simulink model "SYSTEM_MODEL_param_RAMP_SOC"  (R2024a)
settings: Solver=ode45  StartTime=0.0  StopTime=0.5  RelTol=1e-3
undefined symbols (not defined in the file): Cdc, Cf, Co, Dlim, Fsw, Io_max, Ion, kib, kii, kiv, Kmod, kpb, kpi, kpv, L, Lch, Lf, Lithium, Lt, R, Rf, V_grid, Vcv, Vdc
libraries: spsIGBTDiodeLib x7, spsSeriesRLCBranchLib x5, slpidlib x5, spsThreePhaseSeriesRLCBranchLib x3, spsCurrentMeasurementLib x2, spsVoltageMeasurementLib x2, spsabctodq0Lib x2, simulink x1, spsIGBTLib x1, spsPWMGeneratorDCDCLib x1, spsBatteryLib x1, spsPLL3phLib x1
settings Model: Creator=devashishraj  LastModifiedBy=Monz
settings DebuggingCC: UnconnectedInputMsg=warning  UnconnectedOutputMsg=warning  UnconnectedLineMsg=warning
settings ModelReferenceCC: EnableRefExpFcnMdlSchedulingChecks=on
settings RTWCC: GPUComputeCapability=3.5  DLArmComputeVersion=19.05

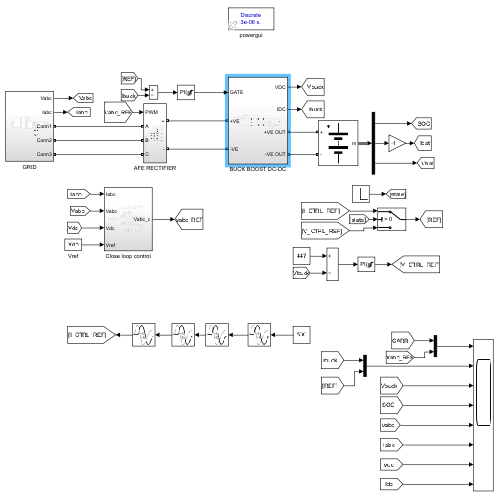
[thumbnail: Simulink's stored preview of the top-level diagram]
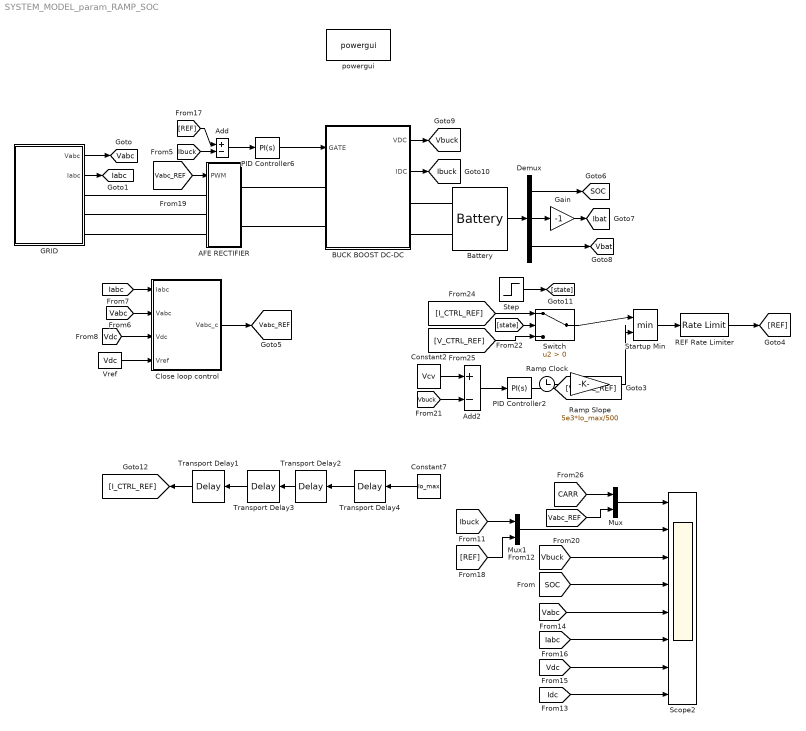
== system SYSTEM_MODEL_param_RAMP_SOC ==
  AFE RECTIFIER : Subsystem
  Add : Sum  Inputs=+-
  Add2 : Sum  Inputs=+-
  BUCK BOOST DC-DC : Subsystem
  Battery : spsBatteryLib/Battery  BatType=Lithium-Ion  ShowTempParam=off  ThermalPreset=no  ShowAgeParam=off  NomV=400  NomQ=250  SOC=SOC0  Batt_Tr=1  PresetModel=on  MaxQ=250  MinV=300  FullV=465.5949  Dis_rate=108.6957  R=0.016  Normal_OP=226.087  expZone="[432.1543      12.28261]"  current=[6.5 13 32.5]  Units=Time  Tci=20  NomT=20  T2=-30  MaxQ2=4.8  FullV2=7.1  Normal_OP2=5.655  expZone2="[6.58           1]"  Rca=0.6  ti=2000  Dp=0  Neq0=0  Tsim=1e6  Ta1=25  Qeol=5.4*0.9  Reol=0.013333*1.2  Char_age=[2.3478, 3]  Dis_age=[2.3478, 10]  N1=1500  N2=10500  N3=1000  N4=1400  Ta2=45  N5=950
  Close loop control : Subsystem
  Constant2 : Constant  Value=Vcv  SampleTime=2e-6
  Constant7 : Constant  Value=Io_max  SampleTime=2e-6
  Demux : Demux  Outputs=3
  GRID : Subsystem
  Gain : Gain  Gain=-1
  Mux : Mux  Inputs=2
  Mux1 : Mux  Inputs=2
  PID Controller2 : slpidlib/PID Controller  Controller=PI  Form=Parallel  TimeDomain=Continuous-time  UseExternalTs=off  SampleTime=-1  IntegratorMethod=Forward Euler  FilterMethod=Forward Euler  ControllerParametersSource=internal  P=0.75  I=50  UseKiTs=off  D=0  UseExternalDerivativeSource=off  N=100  UseFilter=on  TunerSelectOption=Transfer Function Based (PID Tuner App)  ZeroCross=off  InitialConditionSource=internal  InitialConditionForIntegrator=0  InitialConditionForFilter=0  DifferentiatorICPrevScaledInput=0  ExternalReset=none  TrackingMode=off  Kt=1  LimitOutput=on  SatLimitsSource=internal  UpperSaturationLimit=Io_max  LowerSaturationLimit=0  LinearizeAsGain=on  AntiWindupMode=clamping  Kb=1  LimitIntegrator=off  UpperIntegratorSaturationLimit=inf  LowerIntegratorSaturationLimit=-inf  POutMin=[]  POutMax=[]  IOutMin=[]  IOutMax=[]  DOutMin=[]  DOutMax=[]  NOutMin=[]  NOutMax=[]  SumOutMin=[]  SumOutMax=[]  SaturationOutMin=[]  SaturationOutMax=[]  PParamMin=[]  PParamMax=[]  IParamMin=[]  IParamMax=[]  DParamMin=[]  DParamMax=[]  NParamMin=[]  NParamMax=[]  KbParamMin=[]  KbParamMax=[]  KtParamMin=[]  KtParamMax=[]  KbOutMin=[]  KbOutMax=[]  KtOutMin=[]  KtOutMax=[]  IntegratorOutMin=[]  IntegratorOutMax=[]  FilterOutMin=[]  FilterOutMax=[]  SumI1OutMin=[]  SumI1OutMax=[]  SumI2OutMin=[]  SumI2OutMax=[]  SumI3OutMin=[]  SumI3OutMax=[]  SumI4OutMin=[]  SumI4OutMax=[]  SumDOutMin=[]  SumDOutMax=[]  DifferentiatorOutMin=[]  DifferentiatorOutMax=[]  FilterDiffOutCoefMin=[]  FilterDiffOutCoefMax=[]  ReciprocalOutMin=[]  ReciprocalOutMax=[]  SumDenOutMin=[]  SumDenOutMax=[]  SumNumOutMin=[]  SumNumOutMax=[]  DivideOutMin=[]  DivideOutMax=[]  UdiffTsProdOutMin=[]  UdiffTsProdOutMax=[]  NTsProdOutMin=[]  NTsProdOutMax=[]  UintegralTsProdOutMin=[]  UintegralTsProdOutMax=[]  UngainTsProdOutMin=[]  UngainTsProdOutMax=[]  ClampingZeroOutDataTypeStr=Inherit: Inherit via back propagation  ClampingZeroOutMin=[]  ClampingZeroOutMax=[]  FilterDenConstantOutDataTypeStr=Inherit: Inherit via back propagation  FilterDenConstantOutMin=[]  FilterDenConstantOutMax=[]  PCopyOutDataTypeStr=Inherit: Inherit via back propagation  PCopyOutMin=[]  PCopyOutMax=[]  NCopyOutDataTypeStr=Inherit: Inherit via back propagation  NCopyOutMin=[]  NCopyOutMax=[]  IntegratorContinuousStateAttributes=''  IntegratorStateMustResolveToSignalObject=off  IntegratorRTWStateStorageClass=Auto  FilterContinuousStateAttributes=''  FilterStateMustResolveToSignalObject=off  FilterRTWStateStorageClass=Auto  ParallelPVariant=InternalParameters  IdealPVariant=Disabled  IVariant=InternalParameters  DVariant=Disabled  IntegratorVariant=Continuous  SatVariant=Enabled  AWVariant=ContClampingParallel  PCopyVariant=Disabled  TRVariant=Disabled  FdbkBlocksVariant=Forward  IdealPFdbkVariant=Disabled  SatFdbkVariant=Disabled  DerivativeFilterVariant=Disabled  NVariant=Disabled  NCopyVariant=Disabled_SignalSpec  FilterICVariant=Disabled  IntegratorICVariant=InternalICs  ExternalResetVariant=Disabled  TRSumVariant=Passthrough  SumFdbkVariant=Disabled  SumVariant=Sum_PI  TsampFilterVariant=InternalTs  TsampNgainVariant=Passthrough  TsampIntegralVariant=Disabled_SignalSpec  ExternalSaturationOutDataTypeStr=Inherit: Same as second input  DerivativeSourceVariant=Disabled
  PID Controller6 : slpidlib/PID Controller  Controller=PI  Form=Parallel  TimeDomain=Continuous-time  UseExternalTs=off  SampleTime=-1  IntegratorMethod=Forward Euler  FilterMethod=Forward Euler  ControllerParametersSource=internal  P=kpb  I=kib  UseKiTs=off  D=0  UseExternalDerivativeSource=off  N=100  UseFilter=on  TunerSelectOption=Transfer Function Based (PID Tuner App)  ZeroCross=off  InitialConditionSource=internal  InitialConditionForIntegrator=0  InitialConditionForFilter=0  DifferentiatorICPrevScaledInput=0  ExternalReset=none  TrackingMode=off  Kt=1  LimitOutput=on  SatLimitsSource=internal  UpperSaturationLimit=Dlim  LowerSaturationLimit=0  LinearizeAsGain=on  AntiWindupMode=clamping  Kb=1  LimitIntegrator=off  UpperIntegratorSaturationLimit=inf  LowerIntegratorSaturationLimit=-inf  POutMin=[]  POutMax=[]  IOutMin=[]  IOutMax=[]  DOutMin=[]  DOutMax=[]  NOutMin=[]  NOutMax=[]  SumOutMin=[]  SumOutMax=[]  SaturationOutMin=[]  SaturationOutMax=[]  PParamMin=[]  PParamMax=[]  IParamMin=[]  IParamMax=[]  DParamMin=[]  DParamMax=[]  NParamMin=[]  NParamMax=[]  KbParamMin=[]  KbParamMax=[]  KtParamMin=[]  KtParamMax=[]  KbOutMin=[]  KbOutMax=[]  KtOutMin=[]  KtOutMax=[]  IntegratorOutMin=[]  IntegratorOutMax=[]  FilterOutMin=[]  FilterOutMax=[]  SumI1OutMin=[]  SumI1OutMax=[]  SumI2OutMin=[]  SumI2OutMax=[]  SumI3OutMin=[]  SumI3OutMax=[]  SumI4OutMin=[]  SumI4OutMax=[]  SumDOutMin=[]  SumDOutMax=[]  DifferentiatorOutMin=[]  DifferentiatorOutMax=[]  FilterDiffOutCoefMin=[]  FilterDiffOutCoefMax=[]  ReciprocalOutMin=[]  ReciprocalOutMax=[]  SumDenOutMin=[]  SumDenOutMax=[]  SumNumOutMin=[]  SumNumOutMax=[]  DivideOutMin=[]  DivideOutMax=[]  UdiffTsProdOutMin=[]  UdiffTsProdOutMax=[]  NTsProdOutMin=[]  NTsProdOutMax=[]  UintegralTsProdOutMin=[]  UintegralTsProdOutMax=[]  UngainTsProdOutMin=[]  UngainTsProdOutMax=[]  ClampingZeroOutDataTypeStr=Inherit: Inherit via back propagation  ClampingZeroOutMin=[]  ClampingZeroOutMax=[]  FilterDenConstantOutDataTypeStr=Inherit: Inherit via back propagation  FilterDenConstantOutMin=[]  FilterDenConstantOutMax=[]  PCopyOutDataTypeStr=Inherit: Inherit via back propagation  PCopyOutMin=[]  PCopyOutMax=[]  NCopyOutDataTypeStr=Inherit: Inherit via back propagation  NCopyOutMin=[]  NCopyOutMax=[]  IntegratorContinuousStateAttributes=''  IntegratorStateMustResolveToSignalObject=off  IntegratorRTWStateStorageClass=Auto  FilterContinuousStateAttributes=''  FilterStateMustResolveToSignalObject=off  FilterRTWStateStorageClass=Auto  ParallelPVariant=InternalParameters  IdealPVariant=Disabled  IVariant=InternalParameters  DVariant=Disabled  IntegratorVariant=Continuous  SatVariant=Enabled  AWVariant=ContClampingParallel  PCopyVariant=Disabled  TRVariant=Disabled  FdbkBlocksVariant=Forward  IdealPFdbkVariant=Disabled  SatFdbkVariant=Disabled  DerivativeFilterVariant=Disabled  NVariant=Disabled  NCopyVariant=Disabled_SignalSpec  FilterICVariant=Disabled  IntegratorICVariant=InternalICs  ExternalResetVariant=Disabled  TRSumVariant=Passthrough  SumFdbkVariant=Disabled  SumVariant=Sum_PI  TsampFilterVariant=InternalTs  TsampNgainVariant=Passthrough  TsampIntegralVariant=Disabled_SignalSpec  ExternalSaturationOutDataTypeStr=Inherit: Same as second input  DerivativeSourceVariant=Disabled
  Scope2 : Scope  NumInputPorts=8
  Step : Step  Time=0.4  Before=1  After=0  SampleTime=0
  Switch : Switch  Criteria=u2 > Threshold  SaturateOnIntegerOverflow=off  InputSameDT=off
  Transport Delay1 : TransportDelay  DelayTime=0.07  InitialOutput=0.4*Io_max
  Transport Delay2 : TransportDelay  DelayTime=0.07  InitialOutput=0.8*Io_max
  Transport Delay3 : TransportDelay  DelayTime=0.07  InitialOutput=0.6*Io_max
  Transport Delay4 : TransportDelay  DelayTime=0.07  InitialOutput=Io_max
  Vref : Constant  Value=Vdc
  powergui : spspowerguiLib/powergui  Priority=1  SimulationMode=Discrete  SampleTime=3e-6  frequency=60  Iterations=50  frequencyindice=0  Pbase=100e6  ErrMax=1e-4  UnitsV=kV  UnitsW=MW  buscounter=0  FunctionMessages=off  echomessages=off  EnableUseOfTLC=off  CurrentSourceSwitches=off  DisableSnubberDevices=off  DisableRonSwitches=off  DisableVfSwitches=off  DisplayEquations=off  AutomaticDiscreteSolvers=off  SolverType=Tustin/Backward Euler (TBE)  Interpol=off  ExternalGateDelay=off  methode=off  Ts=100  x0status=blocks  SPID=on  SwTol=0  HookPort=off  NonlinearTolerance=1e-4  nMaxIteration=100  ContinueOnMaxIteration=off  RestoreLinks=warning  ResistiveCurrentMeasurement=off  Frange=[0:2:500]  Ylog=off  Xlog=on  ShowGrid=off  save=off  variable=ZData  structure=0  ZoomFFT=off  StartTime=0.0  cycles=1  DisplayStyle=1  fundamental=60  FreqAxis=off  MaxFrequency=1000  frequencyindicesteady=1  RmsSteady=1  display=off
  Ramp Clock : Clock
  Ramp Slope : Gain  Gain=5e3*Io_max/500
  Startup Min : MinMax  Inputs=2
  REF Rate Limiter : RateLimiter  RisingSlewLimit=5e3*Io_max/500  FallingSlewLimit=-(5e3*Io_max/500)
  tag scope: Iabc=global, Ibat=global, Ibuck=global, SOC=global, Vabc=global, Vabc_REF=global, Vbat=global, Vbuck=global
  wires:
  GRID/1(Vabc) -> [Vabc]
  GRID/2(Iabc) -> [Iabc]
  [Iabc] -> Close loop control/1(Iabc)
  [Vabc] -> Close loop control/2(Vabc)
  Battery/1 -> Demux/1
  Demux/2 -> Gain/1
  Demux/1 -> [SOC]
  Gain/1 -> [Ibat]
  Demux/3 -> [Vbat]
  [CARR] -> Mux/1
  Mux/1 -> Scope2/1
  Close loop control/1(Vabc_c) -> [Vabc_REF]
  [Ibuck] -> Add/2
  Add/1 -> PID Controller6/1
  [Ibuck] -> Mux1/1
  Mux1/1 -> Scope2/2
  [SOC] -> Scope2/4
  [Idc] -> Scope2/8
  [Vabc] -> Scope2/5
  [Iabc] -> Scope2/6
  [REF] -> Add/1
  [REF] -> Mux1/2
  [Vabc_REF] -> AFE RECTIFIER/1(PWM)
  [Vabc_REF] -> Mux/2
  PID Controller6/1 -> BUCK BOOST DC-DC/1(GATE)
  BUCK BOOST DC-DC/1(VDC) -> [Vbuck]
  BUCK BOOST DC-DC/2(IDC) -> [Ibuck]
  [state] -> Switch/2
  [V_CTRL_REF] -> Switch/3
  [I_CTRL_REF] -> Switch/1
  Switch/1 -> Startup Min/1
  [Vdc] -> Close loop control/3(Vdc)
  Vref/1 -> Close loop control/4(Vref)
  PID Controller2/1 -> [V_CTRL_REF]
  Add2/1 -> PID Controller2/1
  [Vbuck] -> Add2/2
  Constant2/1 -> Add2/1
  Step/1 -> [state]
  [Vdc] -> Scope2/7
  Constant7/1 -> Transport Delay4/1
  Transport Delay1/1 -> [I_CTRL_REF]
  Transport Delay2/1 -> Transport Delay3/1
  Transport Delay3/1 -> Transport Delay1/1
  Transport Delay4/1 -> Transport Delay2/1
  [Vbuck] -> Scope2/3
  Ramp Clock/1 -> Ramp Slope/1
  Ramp Slope/1 -> Startup Min/2
  Startup Min/1 -> REF Rate Limiter/1
  REF Rate Limiter/1 -> [REF]
  connections:
  GRID/RConn1 -- AFE RECTIFIER/LConn1
  GRID/RConn2 -- AFE RECTIFIER/LConn2
  GRID/RConn3 -- AFE RECTIFIER/LConn3
  BUCK BOOST DC-DC/LConn1 -- AFE RECTIFIER/RConn1
  AFE RECTIFIER/RConn2 -- BUCK BOOST DC-DC/LConn2
  Battery/LConn1 -- BUCK BOOST DC-DC/RConn1
  Battery/LConn2 -- BUCK BOOST DC-DC/RConn2

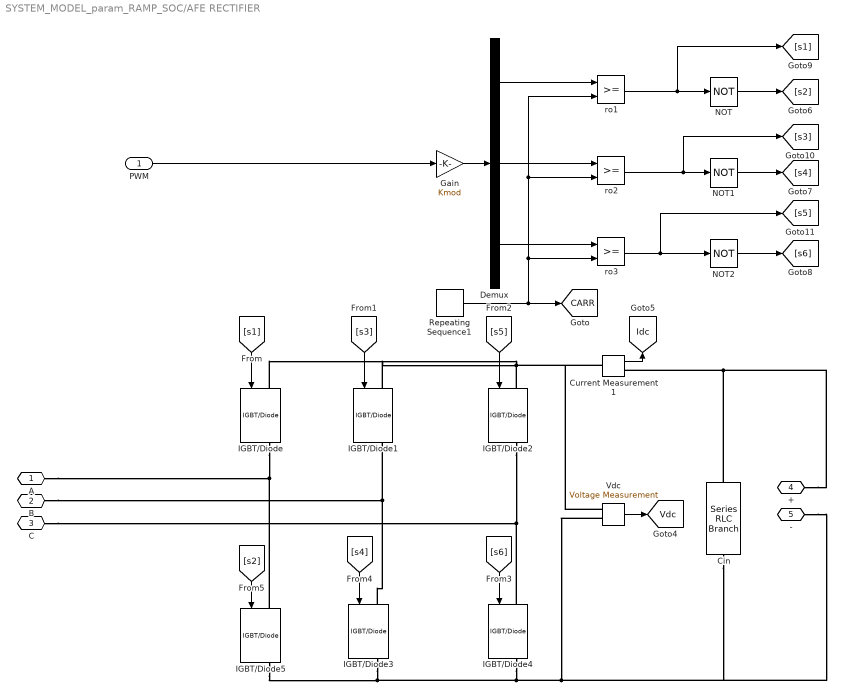
== system SYSTEM_MODEL_param_RAMP_SOC/AFE RECTIFIER ==
  PWM : Inport
  Cin : spsSeriesRLCBranchLib/Series RLC Branch  LConnTagsString=__new0  RConnTagsString=__new0  BranchType=C  Resistance=1  Inductance=1e-3  SetiL0=off  InitialCurrent=0  Capacitance=Cdc  Setx0=off  InitialVoltage=Vdc  Measurements=None
  Current Measurement1 : spsCurrentMeasurementLib/Current Measurement  PhasorSimulation=off  OutputType=Complex  PSBequivalent=0
  Demux : Demux  Outputs=3
  Gain : Gain  Gain=Kmod
  IGBT/Diode{,1..5} (6 alike) : spsIGBTDiodeLib/IGBT//Diode  Ron=1e-3  Rs=1e5  Cs=inf  Measurements=on
  NOT : Logic  Operator=NOT  IconShape=distinctive  AllPortsSameDT=off  OutDataTypeStr=boolean
  NOT1 : Logic  Operator=NOT  IconShape=distinctive  AllPortsSameDT=off  OutDataTypeStr=boolean
  NOT2 : Logic  Operator=NOT  IconShape=distinctive  AllPortsSameDT=off  OutDataTypeStr=boolean
  Repeating Sequence1 : simulink/Sources/Repeating Sequence  rep_seq_t="[0  1/(2*Fsw) 1/Fsw ]"  rep_seq_y=[-1000 1000 -1000]
  Vdc : spsVoltageMeasurementLib/Voltage Measurement  PhasorSimulation=off  OutputType=Complex  PSBequivalent=0
  ro1 : RelationalOperator  OutDataTypeStr=boolean  RndMeth=Simplest  InputSameDT=off
  ro2 : RelationalOperator  OutDataTypeStr=boolean  RndMeth=Simplest  InputSameDT=off
  ro3 : RelationalOperator  OutDataTypeStr=boolean  RndMeth=Simplest  InputSameDT=off
  A : PMIOPort  Side=Left
  B : PMIOPort  Port=2  Side=Left
  C : PMIOPort  Port=3  Side=Left
  + : PMIOPort  Port=4  Side=Right
  - : PMIOPort  Port=5  Side=Right
  tag scope: CARR=global, Idc=global, Vdc=global
  wires:
  NOT2/1 -> [s6]
  Demux/2 -> ro2/1
  PWM/1 -> Gain/1
  [s3] -> IGBT/Diode1/1
  Current Measurement1/1 -> [Idc]
  [s1] -> IGBT/Diode/1
  [s4] -> IGBT/Diode3/1
  Gain/1 -> Demux/1
  Demux/1 -> ro1/1
  [s2] -> IGBT/Diode5/1
  [s5] -> IGBT/Diode2/1
  ro1/1 -> [s1], NOT/1
  ro2/1 -> [s3], NOT1/1
  Demux/3 -> ro3/1
  NOT1/1 -> [s4]
  NOT/1 -> [s2]
  [s6] -> IGBT/Diode4/1
  Vdc/1 -> [Vdc]
  ro3/1 -> [s5], NOT2/1
  Repeating Sequence1/1 -> ro3/2, ro2/2, ro1/2, [CARR]
  connections:
  C/RConn1 -- IGBT/Diode4/LConn1 -- IGBT/Diode2/RConn1
  -/RConn1 -- Cin/RConn1 -- Vdc/LConn2 -- IGBT/Diode5/RConn1 -- IGBT/Diode3/RConn1 -- IGBT/Diode4/RConn1
  Cin/LConn1 -- +/RConn1 -- Current Measurement1/RConn1
  Vdc/LConn1 -- Current Measurement1/LConn1 -- IGBT/Diode2/LConn1 -- IGBT/Diode/LConn1 -- IGBT/Diode1/LConn1
  B/RConn1 -- IGBT/Diode3/LConn1 -- IGBT/Diode1/RConn1
  A/RConn1 -- IGBT/Diode5/LConn1 -- IGBT/Diode/RConn1

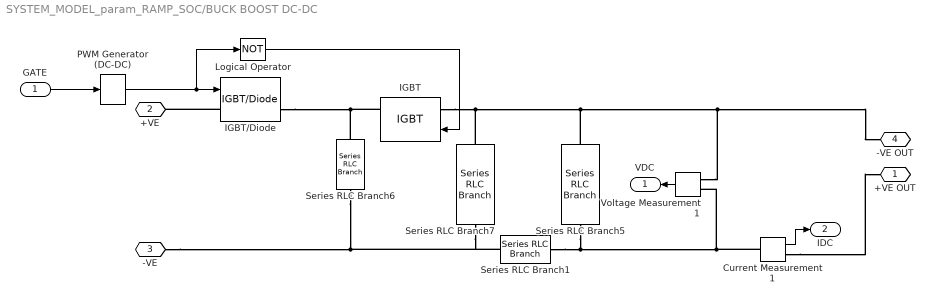
== system SYSTEM_MODEL_param_RAMP_SOC/BUCK BOOST DC-DC ==
  GATE : Inport
  Current Measurement1 : spsCurrentMeasurementLib/Current Measurement  PhasorSimulation=off  OutputType=Complex  PSBequivalent=0
  IGBT : spsIGBTLib/IGBT  Ron=0.001  Lon=0  Vf=1  Tf=1e-6  Tt=2e-6  IC=0  Rs=1e5  Cs=inf  Measurements=on
  IGBT/Diode : spsIGBTDiodeLib/IGBT//Diode  Ron=1e-3  Rs=1e5  Cs=inf  Measurements=on
  Logical Operator : Logic  Operator=NOT  AllPortsSameDT=off  OutDataTypeStr=boolean
  PWM Generator (DC-DC) : spsPWMGeneratorDCDCLib/PWM Generator (DC-DC)  Fsw=100e3  Ts=0
  Series RLC Branch1 : spsSeriesRLCBranchLib/Series RLC Branch  LConnTagsString=__new0  RConnTagsString=__new0  BranchType=L  Resistance=1  Inductance=3e-3  SetiL0=on  InitialCurrent=0  Capacitance=1e-6  Setx0=off  InitialVoltage=0  Measurements=Branch current
  Series RLC Branch5 : spsSeriesRLCBranchLib/Series RLC Branch  LConnTagsString=__new0  RConnTagsString=__new0  BranchType=C  Resistance=1  Inductance=1e-3  SetiL0=off  InitialCurrent=0  Capacitance=Co  Setx0=on  InitialVoltage=0  Measurements=None
  Series RLC Branch6 : spsSeriesRLCBranchLib/Series RLC Branch  LConnTagsString=__new0  RConnTagsString=__new0  BranchType=L  Resistance=1  Inductance=Lch  SetiL0=on  InitialCurrent=0  Capacitance=1e-6  Setx0=off  InitialVoltage=0  Measurements=Branch current
  Series RLC Branch7 : spsSeriesRLCBranchLib/Series RLC Branch  LConnTagsString=__new0  RConnTagsString=__new0  BranchType=C  Resistance=1  Inductance=1e-3  SetiL0=off  InitialCurrent=0  Capacitance=20e-6  Setx0=on  InitialVoltage=0  Measurements=None
  Voltage Measurement1 : spsVoltageMeasurementLib/Voltage Measurement  PhasorSimulation=off  OutputType=Complex  PSBequivalent=0
  +VE OUT : PMIOPort  Side=Right
  +VE : PMIOPort  Port=2  Side=Left
  -VE : PMIOPort  Port=3  Side=Left
  -VE OUT : PMIOPort  Port=4  Side=Right
  VDC : Outport
  IDC : Outport  Port=2
  wires:
  Logical Operator/1 -> IGBT/1
  Current Measurement1/1 -> IDC/1
  GATE/1 -> PWM Generator (DC-DC)/1
  PWM Generator (DC-DC)/1 -> IGBT/Diode/1, Logical Operator/1
  Voltage Measurement1/1 -> VDC/1
  connections:
  IGBT/LConn1 -- Series RLC Branch7/RConn1 -- Series RLC Branch5/RConn1 -- -VE OUT/RConn1 -- Voltage Measurement1/LConn2
  Series RLC Branch5/LConn1 -- Series RLC Branch1/RConn1 -- Voltage Measurement1/LConn1 -- Current Measurement1/LConn1
  Series RLC Branch1/LConn1 -- Series RLC Branch7/LConn1 -- -VE/RConn1 -- Series RLC Branch6/LConn1
  IGBT/RConn1 -- Series RLC Branch6/RConn1 -- IGBT/Diode/RConn1
  IGBT/Diode/LConn1 -- +VE/RConn1
  Current Measurement1/RConn1 -- +VE OUT/RConn1

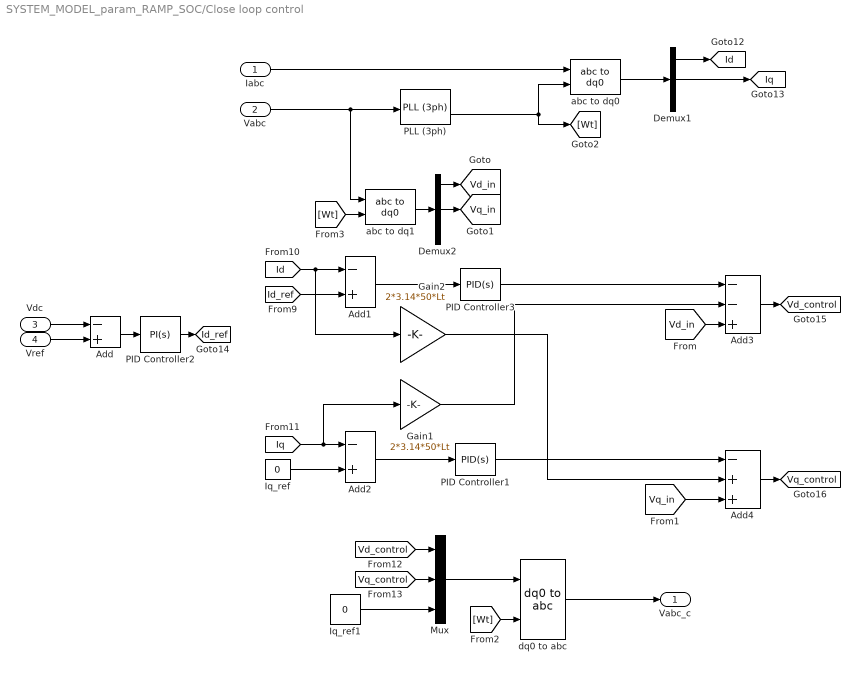
== system SYSTEM_MODEL_param_RAMP_SOC/Close loop control ==
  Iabc : Inport
  Vabc : Inport  Port=2
  Vdc : Inport  Port=3
  Vref : Inport  Port=4
  Add : Sum  Inputs=-+
  Add1 : Sum  Inputs=-+
  Add2 : Sum  Inputs=-+
  Add3 : Sum  Inputs=--+
  Add4 : Sum  Inputs=-++
  Demux1 : Demux  Outputs=3
  Demux2 : Demux  Outputs=3
  Gain1 : Gain  Gain=2*3.14*50*Lt
  Gain2 : Gain  Gain=2*3.14*50*Lt
  Iq_ref : Constant  Value=0
  Iq_ref1 : Constant  Value=0
  Mux : Mux  Inputs=3
  PID Controller1 : slpidlib/PID Controller  Controller=PID  Form=Parallel  TimeDomain=Continuous-time  UseExternalTs=off  SampleTime=-1  IntegratorMethod=Forward Euler  FilterMethod=Forward Euler  ControllerParametersSource=internal  P=kpi  I=kii  UseKiTs=off  D=0  UseExternalDerivativeSource=off  N=100  UseFilter=on  TunerSelectOption=Transfer Function Based (PID Tuner App)  InitialConditionSource=internal  InitialConditionForIntegrator=0  InitialConditionForFilter=0  DifferentiatorICPrevScaledInput=0  ExternalReset=none  TrackingMode=off  Kt=1  LimitOutput=off  SatLimitsSource=internal  UpperSaturationLimit=inf  LowerSaturationLimit=-inf  LinearizeAsGain=on  AntiWindupMode=none  Kb=1  LimitIntegrator=off  UpperIntegratorSaturationLimit=inf  LowerIntegratorSaturationLimit=-inf  POutMin=[]  POutMax=[]  IOutMin=[]  IOutMax=[]  DOutMin=[]  DOutMax=[]  NOutMin=[]  NOutMax=[]  SumOutMin=[]  SumOutMax=[]  SaturationOutMin=[]  SaturationOutMax=[]  PParamMin=[]  PParamMax=[]  IParamMin=[]  IParamMax=[]  DParamMin=[]  DParamMax=[]  NParamMin=[]  NParamMax=[]  KbParamMin=[]  KbParamMax=[]  KtParamMin=[]  KtParamMax=[]  KbOutMin=[]  KbOutMax=[]  KtOutMin=[]  KtOutMax=[]  IntegratorOutMin=[]  IntegratorOutMax=[]  FilterOutMin=[]  FilterOutMax=[]  SumI1OutMin=[]  SumI1OutMax=[]  SumI2OutMin=[]  SumI2OutMax=[]  SumI3OutMin=[]  SumI3OutMax=[]  SumI4OutMin=[]  SumI4OutMax=[]  SumDOutMin=[]  SumDOutMax=[]  DifferentiatorOutMin=[]  DifferentiatorOutMax=[]  FilterDiffOutCoefMin=[]  FilterDiffOutCoefMax=[]  ReciprocalOutMin=[]  ReciprocalOutMax=[]  SumDenOutMin=[]  SumDenOutMax=[]  SumNumOutMin=[]  SumNumOutMax=[]  DivideOutMin=[]  DivideOutMax=[]  UdiffTsProdOutMin=[]  UdiffTsProdOutMax=[]  NTsProdOutMin=[]  NTsProdOutMax=[]  UintegralTsProdOutMin=[]  UintegralTsProdOutMax=[]  UngainTsProdOutMin=[]  UngainTsProdOutMax=[]  ClampingZeroOutDataTypeStr=Inherit: Inherit via back propagation  ClampingZeroOutMin=[]  ClampingZeroOutMax=[]  FilterDenConstantOutDataTypeStr=Inherit: Inherit via back propagation  FilterDenConstantOutMin=[]  FilterDenConstantOutMax=[]  PCopyOutDataTypeStr=Inherit: Inherit via back propagation  PCopyOutMin=[]  PCopyOutMax=[]  NCopyOutDataTypeStr=Inherit: Inherit via back propagation  NCopyOutMin=[]  NCopyOutMax=[]  IntegratorContinuousStateAttributes=''  IntegratorStateMustResolveToSignalObject=off  IntegratorRTWStateStorageClass=Auto  FilterContinuousStateAttributes=''  FilterStateMustResolveToSignalObject=off  FilterRTWStateStorageClass=Auto  ParallelPVariant=InternalParameters  IdealPVariant=Disabled  IVariant=InternalParameters  DVariant=InternalParameters  IntegratorVariant=Continuous  SatVariant=Disabled  AWVariant=Passthrough  PCopyVariant=Disabled  TRVariant=Disabled  FdbkBlocksVariant=Forward  IdealPFdbkVariant=Disabled  SatFdbkVariant=Disabled  DerivativeFilterVariant=ContFilter  NVariant=InternalParameters  NCopyVariant=Disabled  FilterICVariant=InternalICsFilter  IntegratorICVariant=InternalICs  ExternalResetVariant=Disabled  TRSumVariant=Passthrough  SumFdbkVariant=Disabled  SumVariant=Sum_PID  TsampFilterVariant=InternalTs  TsampNgainVariant=Passthrough  TsampIntegralVariant=Disabled_SignalSpec  ExternalSaturationOutDataTypeStr=Inherit: Same as second input  DerivativeSourceVariant=ErrorSignal
  PID Controller2 : slpidlib/PID Controller  Controller=PI  Form=Parallel  TimeDomain=Continuous-time  UseExternalTs=off  SampleTime=2e-6  IntegratorMethod=Forward Euler  FilterMethod=Forward Euler  ControllerParametersSource=internal  P=kpv  I=kiv  UseKiTs=off  D=0  UseExternalDerivativeSource=off  N=100  UseFilter=on  TunerSelectOption=Transfer Function Based (PID Tuner App)  InitialConditionSource=internal  InitialConditionForIntegrator=0  InitialConditionForFilter=0  DifferentiatorICPrevScaledInput=0  ExternalReset=none  TrackingMode=off  Kt=1  LimitOutput=off  SatLimitsSource=internal  UpperSaturationLimit=inf  LowerSaturationLimit=-inf  LinearizeAsGain=on  AntiWindupMode=none  Kb=1  LimitIntegrator=off  UpperIntegratorSaturationLimit=inf  LowerIntegratorSaturationLimit=-inf  POutMin=[]  POutMax=[]  IOutMin=[]  IOutMax=[]  DOutMin=[]  DOutMax=[]  NOutMin=[]  NOutMax=[]  SumOutMin=[]  SumOutMax=[]  SaturationOutMin=[]  SaturationOutMax=[]  PParamMin=[]  PParamMax=[]  IParamMin=[]  IParamMax=[]  DParamMin=[]  DParamMax=[]  NParamMin=[]  NParamMax=[]  KbParamMin=[]  KbParamMax=[]  KtParamMin=[]  KtParamMax=[]  KbOutMin=[]  KbOutMax=[]  KtOutMin=[]  KtOutMax=[]  IntegratorOutMin=[]  IntegratorOutMax=[]  FilterOutMin=[]  FilterOutMax=[]  SumI1OutMin=[]  SumI1OutMax=[]  SumI2OutMin=[]  SumI2OutMax=[]  SumI3OutMin=[]  SumI3OutMax=[]  SumI4OutMin=[]  SumI4OutMax=[]  SumDOutMin=[]  SumDOutMax=[]  DifferentiatorOutMin=[]  DifferentiatorOutMax=[]  FilterDiffOutCoefMin=[]  FilterDiffOutCoefMax=[]  ReciprocalOutMin=[]  ReciprocalOutMax=[]  SumDenOutMin=[]  SumDenOutMax=[]  SumNumOutMin=[]  SumNumOutMax=[]  DivideOutMin=[]  DivideOutMax=[]  UdiffTsProdOutMin=[]  UdiffTsProdOutMax=[]  NTsProdOutMin=[]  NTsProdOutMax=[]  UintegralTsProdOutMin=[]  UintegralTsProdOutMax=[]  UngainTsProdOutMin=[]  UngainTsProdOutMax=[]  ClampingZeroOutDataTypeStr=Inherit: Inherit via back propagation  ClampingZeroOutMin=[]  ClampingZeroOutMax=[]  FilterDenConstantOutDataTypeStr=Inherit: Inherit via back propagation  FilterDenConstantOutMin=[]  FilterDenConstantOutMax=[]  PCopyOutDataTypeStr=Inherit: Inherit via back propagation  PCopyOutMin=[]  PCopyOutMax=[]  NCopyOutDataTypeStr=Inherit: Inherit via back propagation  NCopyOutMin=[]  NCopyOutMax=[]  IntegratorContinuousStateAttributes=''  IntegratorStateMustResolveToSignalObject=off  IntegratorRTWStateStorageClass=Auto  FilterContinuousStateAttributes=''  FilterStateMustResolveToSignalObject=off  FilterRTWStateStorageClass=Auto  ParallelPVariant=InternalParameters  IdealPVariant=Disabled  IVariant=InternalParameters  DVariant=Disabled  IntegratorVariant=Continuous  SatVariant=Disabled  AWVariant=Passthrough  PCopyVariant=Disabled  TRVariant=Disabled  FdbkBlocksVariant=Forward  IdealPFdbkVariant=Disabled  SatFdbkVariant=Disabled  DerivativeFilterVariant=Disabled  NVariant=Disabled  NCopyVariant=Disabled_SignalSpec  FilterICVariant=Disabled  IntegratorICVariant=InternalICs  ExternalResetVariant=Disabled  TRSumVariant=Passthrough  SumFdbkVariant=Disabled  SumVariant=Sum_PI  TsampFilterVariant=InternalTs  TsampNgainVariant=Passthrough  TsampIntegralVariant=Disabled_SignalSpec  ExternalSaturationOutDataTypeStr=Inherit: Same as second input  DerivativeSourceVariant=Disabled
  PID Controller3 : slpidlib/PID Controller  Controller=PID  Form=Parallel  TimeDomain=Continuous-time  UseExternalTs=off  SampleTime=-1  IntegratorMethod=Forward Euler  FilterMethod=Forward Euler  ControllerParametersSource=internal  P=kpi  I=kii  UseKiTs=off  D=0  UseExternalDerivativeSource=off  N=100  UseFilter=on  TunerSelectOption=Transfer Function Based (PID Tuner App)  InitialConditionSource=internal  InitialConditionForIntegrator=0  InitialConditionForFilter=0  DifferentiatorICPrevScaledInput=0  ExternalReset=none  TrackingMode=off  Kt=1  LimitOutput=off  SatLimitsSource=internal  UpperSaturationLimit=inf  LowerSaturationLimit=-inf  LinearizeAsGain=on  AntiWindupMode=none  Kb=1  LimitIntegrator=off  UpperIntegratorSaturationLimit=inf  LowerIntegratorSaturationLimit=-inf  POutMin=[]  POutMax=[]  IOutMin=[]  IOutMax=[]  DOutMin=[]  DOutMax=[]  NOutMin=[]  NOutMax=[]  SumOutMin=[]  SumOutMax=[]  SaturationOutMin=[]  SaturationOutMax=[]  PParamMin=[]  PParamMax=[]  IParamMin=[]  IParamMax=[]  DParamMin=[]  DParamMax=[]  NParamMin=[]  NParamMax=[]  KbParamMin=[]  KbParamMax=[]  KtParamMin=[]  KtParamMax=[]  KbOutMin=[]  KbOutMax=[]  KtOutMin=[]  KtOutMax=[]  IntegratorOutMin=[]  IntegratorOutMax=[]  FilterOutMin=[]  FilterOutMax=[]  SumI1OutMin=[]  SumI1OutMax=[]  SumI2OutMin=[]  SumI2OutMax=[]  SumI3OutMin=[]  SumI3OutMax=[]  SumI4OutMin=[]  SumI4OutMax=[]  SumDOutMin=[]  SumDOutMax=[]  DifferentiatorOutMin=[]  DifferentiatorOutMax=[]  FilterDiffOutCoefMin=[]  FilterDiffOutCoefMax=[]  ReciprocalOutMin=[]  ReciprocalOutMax=[]  SumDenOutMin=[]  SumDenOutMax=[]  SumNumOutMin=[]  SumNumOutMax=[]  DivideOutMin=[]  DivideOutMax=[]  UdiffTsProdOutMin=[]  UdiffTsProdOutMax=[]  NTsProdOutMin=[]  NTsProdOutMax=[]  UintegralTsProdOutMin=[]  UintegralTsProdOutMax=[]  UngainTsProdOutMin=[]  UngainTsProdOutMax=[]  ClampingZeroOutDataTypeStr=Inherit: Inherit via back propagation  ClampingZeroOutMin=[]  ClampingZeroOutMax=[]  FilterDenConstantOutDataTypeStr=Inherit: Inherit via back propagation  FilterDenConstantOutMin=[]  FilterDenConstantOutMax=[]  PCopyOutDataTypeStr=Inherit: Inherit via back propagation  PCopyOutMin=[]  PCopyOutMax=[]  NCopyOutDataTypeStr=Inherit: Inherit via back propagation  NCopyOutMin=[]  NCopyOutMax=[]  IntegratorContinuousStateAttributes=''  IntegratorStateMustResolveToSignalObject=off  IntegratorRTWStateStorageClass=Auto  FilterContinuousStateAttributes=''  FilterStateMustResolveToSignalObject=off  FilterRTWStateStorageClass=Auto  ParallelPVariant=InternalParameters  IdealPVariant=Disabled  IVariant=InternalParameters  DVariant=InternalParameters  IntegratorVariant=Continuous  SatVariant=Disabled  AWVariant=Passthrough  PCopyVariant=Disabled  TRVariant=Disabled  FdbkBlocksVariant=Forward  IdealPFdbkVariant=Disabled  SatFdbkVariant=Disabled  DerivativeFilterVariant=ContFilter  NVariant=InternalParameters  NCopyVariant=Disabled  FilterICVariant=InternalICsFilter  IntegratorICVariant=InternalICs  ExternalResetVariant=Disabled  TRSumVariant=Passthrough  SumFdbkVariant=Disabled  SumVariant=Sum_PID  TsampFilterVariant=InternalTs  TsampNgainVariant=Passthrough  TsampIntegralVariant=Disabled_SignalSpec  ExternalSaturationOutDataTypeStr=Inherit: Same as second input  DerivativeSourceVariant=ErrorSignal
  PLL (3ph) : spsPLL3phLib/PLL (3ph)  Fmin=45  Par_Init=[0, 60]  ParK=[180, 3200, 1]  TcD=1e-4  MaxRateChangeFreq=12  FilterCutOffFreq=25  Ts=0  AGC=on
  abc to dq0 : spsabctodq0Lib/abc to dq0  Alignment=90 degrees behind phase A axis
  abc to dq1 : spsabctodq0Lib/abc to dq0  Alignment=90 degrees behind phase A axis
  dq0 to abc : spsdq0toabcLib/dq0 to abc  Alignment=90 degrees behind phase A axis
  Vabc_c : Outport
  tag scope: Id=global, Id_ref=global, Iq=global, Vd_control=global, Vd_in=global, Vq_control=global, Vq_in=global
  wires:
  Demux1/1 -> [Id]
  Add2/1 -> PID Controller1/1
  [Vd_control] -> Mux/1
  [Id_ref] -> Add1/2
  Iabc/1 -> abc to dq0/1
  [Iq] -> Gain1/1, Add2/1
  Vabc/1 -> abc to dq1/1, PLL (3ph)/1
  [Id] -> Gain2/1, Add1/1
  abc to dq0/1 -> Demux1/1
  Add3/1 -> [Vd_control]
  Demux1/2 -> [Iq]
  [Vq_control] -> Mux/2
  Iq_ref/1 -> Add2/2
  Iq_ref1/1 -> Mux/3
  Add4/1 -> [Vq_control]
  PLL (3ph)/2 -> [Wt], abc to dq0/2
  Mux/1 -> dq0 to abc/1
  Add1/1 -> PID Controller3/1
  Gain1/1 -> Add3/2
  abc to dq1/1 -> Demux2/1
  Demux2/1 -> [Vd_in]
  Demux2/2 -> [Vq_in]
  [Vd_in] -> Add3/3
  Gain2/1 -> Add4/2
  [Vq_in] -> Add4/3
  dq0 to abc/1 -> Vabc_c/1
  PID Controller3/1 -> Add3/1
  PID Controller1/1 -> Add4/1
  [Wt] -> dq0 to abc/2
  [Wt] -> abc to dq1/2
  PID Controller2/1 -> [Id_ref]
  Vdc/1 -> Add/1
  Vref/1 -> Add/2
  Add/1 -> PID Controller2/1

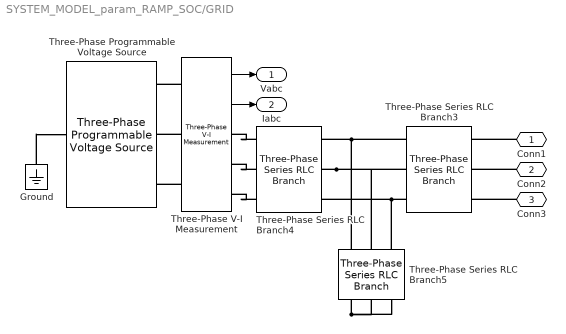
== system SYSTEM_MODEL_param_RAMP_SOC/GRID ==
  Ground : spsGroundLib/Ground  LConnTagsString=a
  Three-Phase Programmable Voltage Source : spsThreePhaseProgrammableVoltageSourceLib/Three-Phase Programmable Voltage Source  PositiveSequence="[V_grid  0 50]"  VariationEntity=None  VariationType=Table of time-amplitude pairs  VariationTypeAlt=Step  VariationStep=0.5  VariationRate=10  VariationMagnitude=0.3  VariationFrequency=2  VariationTiming=[1 2]  VariationPhaseA=off  Amplitudes=[1 0.8 1.2 1.0]  TimeValues=[0 0.1 0.15 0.2]  HarmonicGeneration=off  HarmonicA=[3 0.2 -25 0]  HarmonicB=[2 0.15 35 2]  Timing="[0.05  3]"  BusType=swing  Pref=0  Qref=0  Qmin=-inf  Qmax=inf
  Three-Phase Series RLC Branch3 : spsThreePhaseSeriesRLCBranchLib/Three-Phase Series RLC Branch  LConnTagsString=A|B|C  RConnTagsString=A|B|C  BranchType=RL  Resistance=R  Inductance=L  Capacitance=1e-6  Measurements=None
  Three-Phase Series RLC Branch4 : spsThreePhaseSeriesRLCBranchLib/Three-Phase Series RLC Branch  LConnTagsString=A|B|C  RConnTagsString=A|B|C  BranchType=RL  Resistance=Rf  Inductance=Lf  Capacitance=1e-6  Measurements=None
  Three-Phase Series RLC Branch5 : spsThreePhaseSeriesRLCBranchLib/Three-Phase Series RLC Branch  LConnTagsString=A|B|C  RConnTagsString=A|B|C  BranchType=RC  Resistance=2  Inductance=150e-6  Capacitance=Cf  Measurements=None
  Three-Phase V-I Measurement : spsThreePhaseVIMeasurementLib/Three-Phase V-I Measurement  VoltageMeasurement=phase-to-ground  SetLabelV=off  LabelV=Vabc  Vpu=off  VpuLL=off  CurrentMeasurement=yes  SetLabelI=off  LabelI=Iabc  Ipu=off  Pbase=100e6  Vbase=500e3  OutputType=Complex  PhasorSimulation=off  PSBequivalent=0
  Conn1 : PMIOPort  Side=Right
  Conn2 : PMIOPort  Port=2  Side=Right
  Conn3 : PMIOPort  Port=3  Side=Right
  Vabc : Outport
  Iabc : Outport  Port=2
  wires:
  Three-Phase V-I Measurement/1 -> Vabc/1
  Three-Phase V-I Measurement/2 -> Iabc/1
  connections:
  Three-Phase V-I Measurement/LConn1 -- Three-Phase Programmable Voltage Source/RConn1
  Three-Phase V-I Measurement/LConn3 -- Three-Phase Programmable Voltage Source/RConn3
  Three-Phase V-I Measurement/LConn2 -- Three-Phase Programmable Voltage Source/RConn2
  Ground/LConn1 -- Three-Phase Programmable Voltage Source/LConn1
  Three-Phase Series RLC Branch4/LConn2 -- Three-Phase Series RLC Branch5/LConn2 -- Three-Phase Series RLC Branch3/RConn2
  Three-Phase Series RLC Branch3/RConn3 -- Three-Phase Series RLC Branch4/LConn3 -- Three-Phase Series RLC Branch5/LConn3
  Three-Phase Series RLC Branch5/LConn1 -- Three-Phase Series RLC Branch4/LConn1 -- Three-Phase Series RLC Branch3/RConn1
  Three-Phase Series RLC Branch5/RConn1 -- Three-Phase Series RLC Branch5/RConn2 -- Three-Phase Series RLC Branch5/RConn3
  Conn3/RConn1 -- Three-Phase Series RLC Branch3/LConn3
  Conn1/RConn1 -- Three-Phase Series RLC Branch3/LConn1
  Conn2/RConn1 -- Three-Phase Series RLC Branch3/LConn2
  Three-Phase Series RLC Branch4/RConn1 -- Three-Phase V-I Measurement/RConn1
  Three-Phase Series RLC Branch4/RConn2 -- Three-Phase V-I Measurement/RConn2
  Three-Phase Series RLC Branch4/RConn3 -- Three-Phase V-I Measurement/RConn3
